simulink model "PalletizeBoxesUsingCobot"  (R2025b)
settings: Solver=FixedStepDiscrete  StartTime=0.0  StopTime=inf  FixedStep=0.01  RelTol=1e-3
PreLoadFcn:
  | EnableGeospatial = false;
  | assignin("base","EnableGeospatial",EnableGeospatial);
  | projectDir = fileparts(which('PalletizeBoxesUsingCobot.slx'));
  | if projectDir == ""
  |     projectDir = pwd;
  | end
  | BoxSet = readtable(fullfile(projectDir,"boxes.xlsx"));
  | assignin("base","BoxSet",BoxSet);
InitFcn:
  | clear boxData boxDataAll boxTable layoutPlan layoutPos layoutYaw layoutH layoutN boxDim boxWeight boxPosition pickPosition boxToEEOffset suctionCenterOffsetCheck maxNumOfBoxes executionActionLog executionActorRegistry
  | projectDir = fileparts(which('PalletizeBoxesUsingCobot.slx'));
  | if projectDir == ""
  |     projectDir = pwd;
  | end
  | disp("Reading Excel from: " + fullfile(projectDir,"boxes.xlsx"));
  | boxTable = readtable(fullfile(projectDir,"boxes.xlsx"));
  | cfg = palletTaskConfig();
  | EnableGeospatial = false;
  | boxDataAll.length = boxTable.L;
  | boxDataAll.width  = boxTable.W;
  | boxDataAll.height = boxTable.H;
  | boxDataAll.weight = boxTable.Mass;
  | if ismember("Type", string(boxTable.Properties.VariableNames)); boxDataAll.type = string(boxTable.Type); end
  | layoutBoxOffset = cfg.layoutBoxOffset;
  | firstExcelID = cfg.firstExcelID;
  | boxData = sliceBoxData(boxDataAll, firstExcelID);
  | nLayoutBoxes = min(cfg.maxLayoutBoxes, numel(boxData.length));
  | boxData.length = boxData.length(1:nLayoutBoxes);
  | boxData.width = boxData.width(1:nLayoutBoxes);
  | boxData.height = boxData.height(1:nLayoutBoxes);
  | boxData.weight = boxData.weight(1:nLayoutBoxes);
  | if isfield(boxData,"type"); boxData.type = boxData.type(1:nLayoutBoxes); end
  | palletDim = cfg.palletDim;
  | palletMargin = cfg.palletMargin;
  | boxGap = cfg.boxGap;
  | palletLoc = cfg.palletLoc;
  | batchSize = cfg.batchSize;
  | layoutPlan = buildLayoutPlanBatch3(boxData, palletDim, palletLoc, batchSize, palletMargin, boxGap);
  | executionPlan = buildBufferExecutionPlan(layoutPlan, cfg);
  | layoutN = numel(layoutPlan);
  | layoutPos = zeros(layoutN,3);
  | layoutYaw = zeros(layoutN,1);
  | layoutH = zeros(layoutN,1);
  | for i = 1:layoutN
  |     layoutPos(i,:) = layoutPlan(i).pos;
  |     layoutYaw(i) = layoutPlan(i).yaw;
  |     layoutH(i) = layoutPlan(i).H;
  | end
  | boxDim = [boxData.length(1); boxData.width(1); boxData.height(1)];
  | boxWeight = boxData.weight(1);
  | boxPosition = cfg.sourceBoxPosition;
  | pickPosition = cfg.pickPosition;
  | boxToEEOffset = [-0.2 0 boxDim(3)/2 + 0.11];
  | suctionCenterOffsetCheck = boxToEEOffset + [0.2 0 0];
  | maxNumOfBoxes = numel(executionPlan);
  | enableSimulinkRRT = false;
  | executionActionLog = zeros(0,4);
  | executionActorRegistry = cell(1,layoutN);
  | rbt = exampleHelperSetUpCobot();
  | assignin("base","boxData",boxData);
  | assignin("base","boxDataAll",boxDataAll);
  | assignin("base","layoutBoxOffset",layoutBoxOffset);
  | assignin("base","firstExcelID",firstExcelID);
  | assignin("base","palletDim",palletDim);
  | assignin("base","palletMargin",palletMargin);
  | assignin("base","boxGap",boxGap);
  | assignin("base","palletLoc",palletLoc);
  | assignin("base","layoutPlan",layoutPlan);
  | assignin("base","executionPlan",executionPlan);
  | assignin("base","layoutMethod","Constructive");
  | assignin("base","batchSize",batchSize);
  | assignin("base","layoutPos",layoutPos);
  | assignin("base","layoutYaw",layoutYaw);
  | assignin("base","layoutH",layoutH);
  | assignin("base","layoutN",layoutN);
  | assignin("base","boxDim",boxDim);
  | assignin("base","boxWeight",boxWeight);
  | assignin("base","boxPosition",boxPosition);
  | assignin("base","pickPosition",pickPosition);
  | assignin("base","boxToEEOffset",boxToEEOffset);
  | assignin("base","suctionCenterOffsetCheck",suctionCenterOffsetCheck);
  | assignin("base","maxNumOfBoxes",maxNumOfBoxes);
  | assignin("base","enableSimulinkRRT",enableSimulinkRRT);
  | assignin("base","executionActionLog",executionActionLog);
  | assignin("base","executionActorRegistry",executionActorRegistry);
  | assignin("base","rbt",rbt);
  | assignin("base","EnableGeospatial",EnableGeospatial);
StartFcn:
  | coder.extrinsic("spawnBox")
  | coder.extrinsic("spawnBufferZone")
  | coder.extrinsic("selectBoxDim")
  | [boxDim, boxWeight] = selectBoxDim(0);
  | boxToEEOffset = [-0.2 0 boxDim(3)/2 + 0.11];
  | suctionCenterOffsetCheck = boxToEEOffset + [0.2 0 0];
  | assignin("base","boxDim",boxDim);
  | assignin("base","boxWeight",boxWeight);
  | assignin("base","boxToEEOffset",boxToEEOffset);
  | assignin("base","suctionCenterOffsetCheck",suctionCenterOffsetCheck);
  | spawnBufferZone()
  | spawnBox(0,boxPosition,boxDim)
StopFcn:
  | try
  |     if exist("executionPlan","var") && ~isempty(executionPlan)
  |         finalizeExecutionAction(numel(executionPlan)-1);
  |     end
  | catch ME
  |     warning("PalletizeBoxes:FinalizeLastAction","%s",ME.message);
  | end
  | disp("Buffer execution simulation stopped.")
libraries: sim3dlib x2, robotcorelib x2, robotmaniplib x2, robotsim3dlib x1, simulink x1
settings Model: PauseTimes=1  Creator=araman  LastModifiedBy=周家易1
settings DebuggingCC: ReadBeforeWriteMsg=DisableAll  WriteAfterWriteMsg=DisableAll  WriteAfterReadMsg=DisableAll  MultiTaskDSMMsg=none
settings ModelReferenceCC: UpdateModelReferenceTargets=IfOutOfDate
settings SFSimCC: SFSimEcho=off

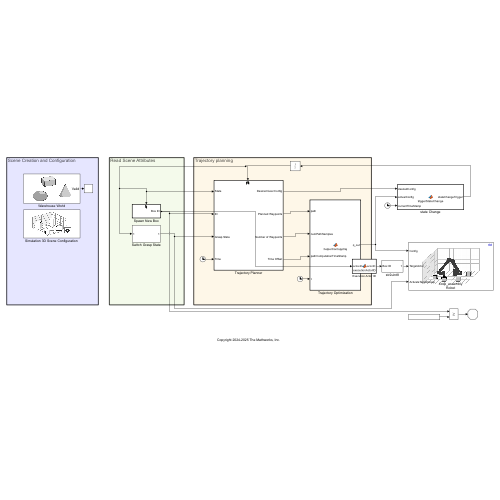
[thumbnail: Simulink's stored preview of the top-level diagram]
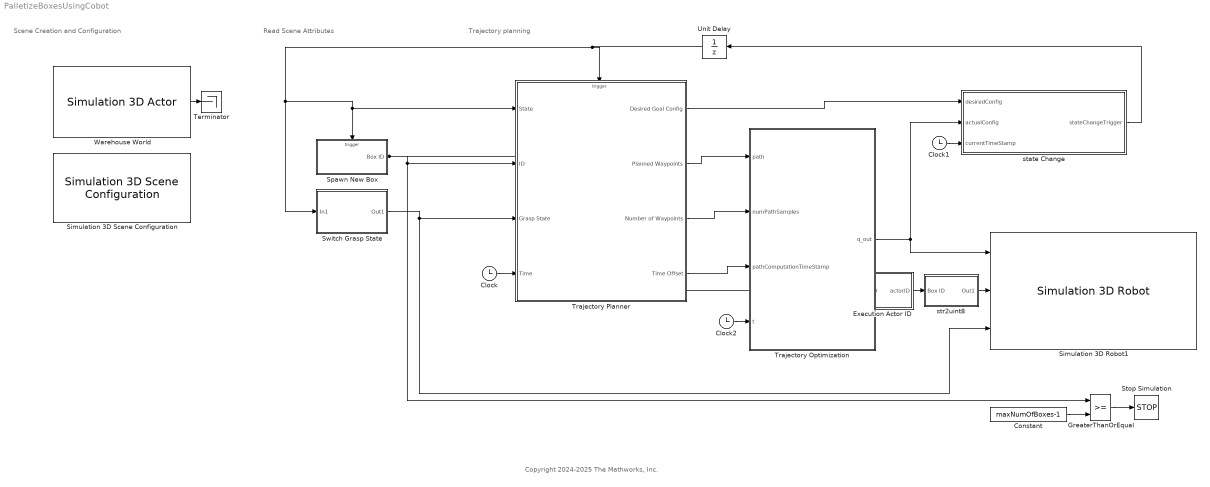
== system PalletizeBoxesUsingCobot ==
  note: Copyright 2024-2025 The Mathworks, Inc.
  note: Trajectory planning
  note: Scene Creation and Configuration
  note: Read Scene Attributes
  Clock : Clock
  Clock1 : Clock
  Clock2 : Clock
  Constant : Constant  Value=maxNumOfBoxes-1
  Execution Actor ID : MATLAB Function  TreatAsAtomicUnit=on
  GreaterThanOrEqual : RelationalOperator  OutDataTypeStr=boolean  RndMeth=Simplest  InputSameDT=off
  Simulation 3D Robot1 : robotsim3dlib/Simulation 3D Robot  actorInputType=RigidBodyTree Object  RigidBodyTree=rbt  ActorName=Robot  existActorChekBox=off  initialTrans=[0 0 0]  initialRot=[0 0 0]  initialConfig="[2.8471   -1.6598    2.1329    4.2393   -1.5708    4.4179]"  EndEffector=4cup_assembly  eeOffsetInpChekBox=off  eeTargetTrans=[0 -0.2 0]  eeTargetRot=[0 0 0]  enableRegionGraspChekBox=off  regionGraspInpChekBox=off  eeTargTransDiff=[0.2 0.2 0.2]  eeTargRotDiff=[0 0 0]  enableVisualVisualization=on  enableCollisionVisualization=off  collisionGeomColor=[0 1 0]  collisionGeomTransp=0.1  inpConfEnbVal=on  inpGraspEnbVal=on  inpTransEnbVal=off  outConfEnbVal=off  outGraspEnbVal=off  outTransEnbVal=off  SampleTime=-1  ActorType=SimulinkVehicle  ID=C  aMode=6  ActorTag=Robot  Mesh=RigidBodyTree
  "Simulation 3D Scene Configuration " : sim3dlib/Simulation 3D Scene Configuration  Priority=0  ProjectFormat=Default Scenes  SceneDesc=Empty scene  ProjectName=D:\matlab2025b\toolbox\shared\sim3d_projects\automotive_project_windows\UE\WindowsNoEditor\VehicleSimulation.exe  ScenePath=/Game/Maps/EmptyScene  EnableOpenDRIVE=off  vehTagList={'Custom';'Robot';'Scene Origin';'Warehouse'}  vehTag=Robot  AttachedCameraRelativeTranslation=[0 0 0]  FreeCameraDefaultInitialTranslation=[-6, 0, 2]  AttachedCameraRelativeRotation=[0 0 0]  FreeCameraDefaultInitialRotation=[0, -15, 0]  ViewpointName=Custom  FreeCameraInitialTranslation=[0, 0, 5]  ViewpointTranslation=[0 0 0]  FreeCameraInitialRotation=[0, -90, 0]  ViewpointRotation=[0 0 0]  OpVisEn=off  Ts=0.02  EnableWindow=on  EnableRemoteAccess=off  EnableWeather=off  SunAzimuth=90  SunAltitude=40.0  EnableGeospatialSun=off  Latitude=0  Longitude=0  Date=2023-01-01  Time=10:30:00  GeoTimeZone=-5.0  SunDaylightSaving=off  wind=1  clouds=10  EnableVolumetricClouds=off  CloudCoverage=0  CloudAltitude=6  fog=0  rain=0  RaindropsEffect=off  SnowDensity=0  EnableGeospatial=off  TilesetSource=Earth terrain  UseTrueOrigin=off  OriginHeight=200  OriginLatitude=40.744652  OriginLongitude=-73.988864  MapStyle=Aerial  AdditionalAssetIDs=[]  UseAdvancedSunSky=off  SolarTime=11  TimeZone=-5  Day=21  Month=9  Year=2022  UseDaylightSavingTime=on  DSTStartDay=10  DSTStartMonth=3  DSTEndDay=3  DSTEndMonth=11  DSTSwitchHour=2  sensorTag=MainCamera2  sensorId=2  sensorName=MainCamera2  mountLoc=Origin  offsetFlag=off  tmountOffset=[0, 0, 0]  rmountOffset=[0, 0, 0]  HorizontalResolution=1280  VerticalResolution=720  HorizontalFOV=60  mountPoint=[0 0 0]  mountOrientation=[0 0 0]  aMode=6  ID=2  GeoTrigger=Inactive  ViewNameList={'Custom'}  ViewTranslationList={'[0 0 5]'}  ViewRotationList={'[0 -90 0]'}
      settings: LibrarySourceBlock=robotsim3dlib/Simulation 3D Scene Configuration
  Spawn New Box : Subsystem  TreatAsAtomicUnit=on
  Stop Simulation : Stop
  Switch Grasp State : Subsystem
  Terminator : Terminator
  Trajectory Optimization : MATLAB Function  TreatAsAtomicUnit=on
  Trajectory Planner : Subsystem
  Unit Delay : UnitDelay  InitialCondition=-1  SampleTime=-1  HasFrameUpgradeWarning=on
  Warehouse World : sim3dlib/Simulation 3D Actor  Priority=1  ActorName=Warehouse  ParentName=Scene Origin  Operation=Create at setup  InitScriptText=|  SampleTime=-1  Translation=single([0 0 0])  Rotation=single([0 0 0])  Scale=single([1 1 1])  aMode=5  ActorTag=Warehouse  ActorType=Sim3dActor  ID=2
      | Plane = sim3d.Actor(ActorName='Plane');
      | Plane.createShape('plane',[5 5 0.1]);
      | Plane.PreciseContacts = true;
      | Plane.Color = [81, 94, 120]/256;
      | add(World,Plane,Actor);
      | 
      | Base = sim3d.Actor('ActorName','collBase');
      | Base.createShape('box',[0.25,0.25,0.5]);
      | Base.Translation = [0,0,0.25];
      | Base.Color = [87, 67, 60]/256;
      | add(World,Base,Actor);
      | 
      | Bench = sim3d.Actor('ActorName','collBench');
      | Bench.createShape('box',[0.8 0.8 0.5]);
      | Bench.Translation = [-0.7 -0.7 0.25];
      | Bench.Color = [87, 67, 60]/256;
      | add(World,Bench,Actor);
      | 
      | Pallet = sim3d.Actor(ActorName='collPallet');
      | add(World,Pallet,Actor)
      | load(Pallet,"PalletEuro.stl",0.001*[1 1 1]);
      | Pallet.Translation = [-1 -0.3 0];
      | Pallet.Collisions = true;
      | Pallet.PreciseContacts = true;
      | PalletDeck = sim3d.Actor(ActorName='PalletDeck');
      | PalletDeck.createShape('box',[0.8 1.2 0.01]);
      | PalletDeck.Translation = [-0.6 0.3 0.139];
      | PalletDeck.Collisions = true;
      | PalletDeck.PreciseContacts = true;
      | PalletDeck.Color = [1 1 1];
      | try, PalletDeck.Opacity = 0; catch, end
      | try, PalletDeck.Transparency = 1; catch, end
      | try, PalletDeck.Visible = false; catch, end
      | add(World,PalletDeck,Actor);
      | 
      | 
      | 
      | 
      | 
      | 
      | 
      | 
      | 
      | 
      | 
      | 
      | 
      | 
      | 
      | 
      | 
      | 
      | 
      | 
      | 
      | 
      | 
      | 
      | 
      | 
      | 
      | Pallet.Collisions = true;
      | Pallet.PreciseContacts = true;
      | Pallet.Collisions = true;
      | Pallet.PreciseContacts = true;
      | Pallet.Collisions = true;
      | Pallet.PreciseContacts = true;
      | Pallet.Collisions = true;
      | Pallet.PreciseContacts = true;
      | Pallet.Collisions = true;
      | Pallet.PreciseContacts = true;
      | Pallet.Collisions = true;
      | Pallet.PreciseContacts = true;
      | Pallet.Collisions = true;
      | Pallet.PreciseContacts = true;
      | Pallet.Collisions = true;
      | Pallet.PreciseContacts = true;
      | Pallet.Collisions = true;
      | Pallet.PreciseContacts = true;
      | Pallet.Collisions = true;
      | Pallet.PreciseContacts = true;
      | Pallet.Collisions = true;
      | Pallet.PreciseContacts = true;
      | Pallet.Collisions = true;
      | Pallet.PreciseContacts = true;
      | Pallet.Collisions = true;
      | Pallet.PreciseContacts = true;
  state Change : MATLAB Function  TreatAsAtomicUnit=on
  str2uint8 : Subsystem
  wires:
  Warehouse World/1 -> Terminator/1
  Unit Delay/1 -> Switch Grasp State/1(In1), Spawn New Box/Trigger, Trajectory Planner/1(State), Trajectory Planner/Trigger
  Clock/1 -> Trajectory Planner/4(Time)
  Trajectory Planner/2(Planned Waypoints) -> Trajectory Optimization/1(path)
  Trajectory Planner/3(Number of Waypoints) -> Trajectory Optimization/2(numPathSamples)
  Trajectory Planner/4(Time Offset) -> Trajectory Optimization/3(pathComputationTimeStamp)
  Trajectory Planner/1(Desired Goal Config) -> state Change/1(desiredConfig)
  Spawn New Box/1(Box ID) -> Trajectory Planner/2(ID), GreaterThanOrEqual/1, Execution Actor ID/1(actionID)
  Clock1/1 -> state Change/3(currentTimeStamp)
  state Change/1(stateChangeTrigger) -> Unit Delay/1
  Clock2/1 -> Trajectory Optimization/4(t)
  Switch Grasp State/1(Out1) -> Simulation 3D Robot1/3, Trajectory Planner/3(Grasp State)
  Trajectory Optimization/1(q_out) -> Simulation 3D Robot1/1, state Change/2(actualConfig)
  Constant/1 -> GreaterThanOrEqual/2
  GreaterThanOrEqual/1 -> Stop Simulation/1
  str2uint8/1(Out1) -> Simulation 3D Robot1/2
  Execution Actor ID/1(actorID) -> str2uint8/1(Box ID)

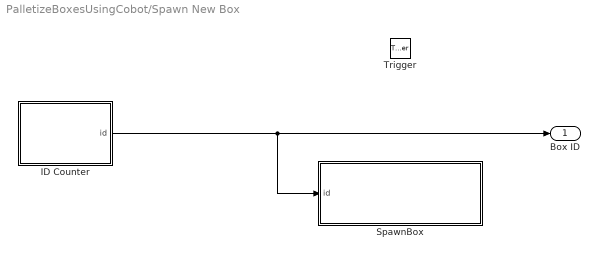
== system PalletizeBoxesUsingCobot/Spawn New Box ==
  Trigger : TriggerPort  TriggerType=falling  VariantControl=(inherit)
  ID Counter : Subsystem
  "SpawnBox " : MATLAB Function  TreatAsAtomicUnit=on
  Box ID : Outport
  wires:
  ID Counter/1(id) -> "SpawnBox "/1(id), Box ID/1

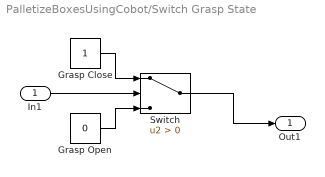
== system PalletizeBoxesUsingCobot/Switch Grasp State ==
  In1 : Inport
  Grasp Close : Constant  OutDataTypeStr=boolean
  Grasp Open : Constant  Value=0  OutDataTypeStr=boolean
  Switch : Switch  Criteria=u2 > Threshold  SaturateOnIntegerOverflow=off  InputSameDT=off
  Out1 : Outport
  wires:
  Grasp Close/1 -> Switch/1
  Switch/1 -> Out1/1
  Grasp Open/1 -> Switch/3
  In1/1 -> Switch/2

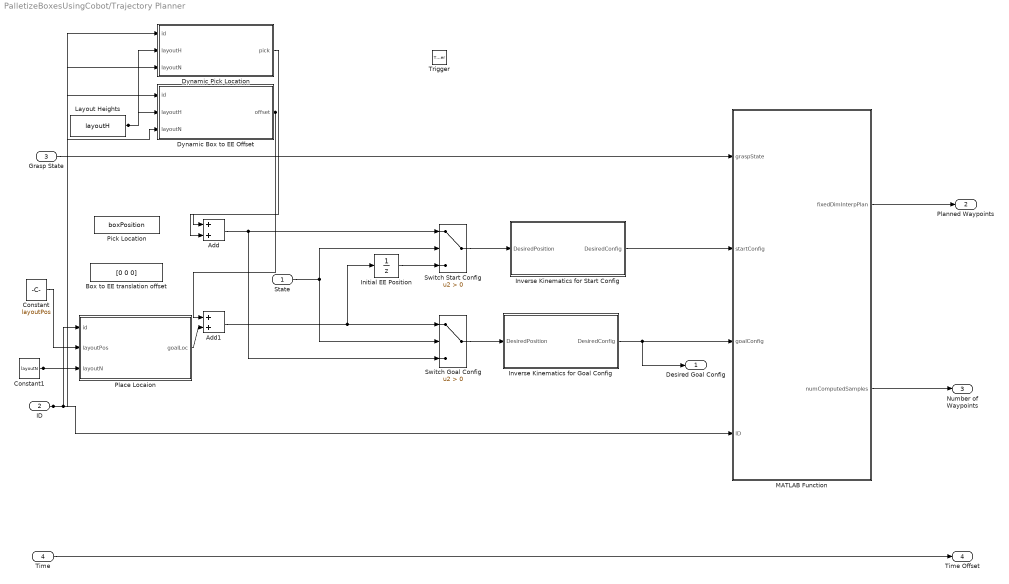
== system PalletizeBoxesUsingCobot/Trajectory Planner ==
  State : Inport
  ID : Inport  Port=2
  Grasp State : Inport  Port=3
  Time : Inport  Port=4
  Trigger : TriggerPort  TriggerType=either  VariantControl=(inherit)  OutputDataType=double  InitialTriggerSignalState=zero  PortDimensions=1
  Add : Sum
  Add1 : Sum
  Box to EE translation offset : Constant  Value=[0 0 0]  VectorParams1D=off
  Constant : Constant  Value=layoutPos
  Constant1 : Constant  Value=layoutN
  Dynamic Box to EE Offset : MATLAB Function  TreatAsAtomicUnit=on
  Dynamic Pick Location : MATLAB Function  TreatAsAtomicUnit=on
  Initial EE Position : UnitDelay  InitialCondition=[-0.6 0 0.8]  SampleTime=-1  HasFrameUpgradeWarning=on
  Inverse Kinematics for Goal Config : Subsystem
  Inverse Kinematics for Start Config : Subsystem
  Layout Heights : Constant  Value=layoutH
  MATLAB Function : MATLAB Function  TreatAsAtomicUnit=on
  Pick Location : Constant  Value=boxPosition  VectorParams1D=off
  Place Locaion : MATLAB Function  TreatAsAtomicUnit=on
  Switch Goal Config : Switch  Criteria=u2 > Threshold  SaturateOnIntegerOverflow=off  InputSameDT=off
  Switch Start Config : Switch  Criteria=u2 > Threshold  SaturateOnIntegerOverflow=off  InputSameDT=off
  Desired Goal Config : Outport
  Planned Waypoints : Outport  Port=2
  Number of Waypoints : Outport  Port=3
  Time Offset : Outport  Port=4
  wires:
  MATLAB Function/1(fixedDimInterpPlan) -> Planned Waypoints/1
  MATLAB Function/2(numComputedSamples) -> Number of Waypoints/1
  Inverse Kinematics for Start Config/1(DesiredConfig) -> MATLAB Function/2(startConfig)
  Inverse Kinematics for Goal Config/1(DesiredConfig) -> MATLAB Function/3(goalConfig), Desired Goal Config/1
  Time/1 -> Time Offset/1
  Switch Start Config/1 -> Inverse Kinematics for Start Config/1(DesiredPosition)
  Initial EE Position/1 -> Switch Start Config/3
  Switch Goal Config/1 -> Inverse Kinematics for Goal Config/1(DesiredPosition)
  Add/1 -> Switch Start Config/1, Switch Goal Config/3
  State/1 -> Switch Start Config/2, Switch Goal Config/2
  Grasp State/1 -> MATLAB Function/1(graspState)
  ID/1 -> MATLAB Function/4(ID), Place Locaion/1(id), Dynamic Box to EE Offset/1(id), Dynamic Pick Location/1(id)
  Place Locaion/1(goalLoc) -> Add1/2
  Add1/1 -> Initial EE Position/1, Switch Goal Config/1
  Constant/1 -> Place Locaion/2(layoutPos)
  Constant1/1 -> Place Locaion/3(layoutN), Dynamic Box to EE Offset/3(layoutN), Dynamic Pick Location/3(layoutN)
  Layout Heights/1 -> Dynamic Box to EE Offset/2(layoutH), Dynamic Pick Location/2(layoutH)
  Dynamic Box to EE Offset/1(offset) -> Add/2, Add1/1
  Dynamic Pick Location/1(pick) -> Add/1

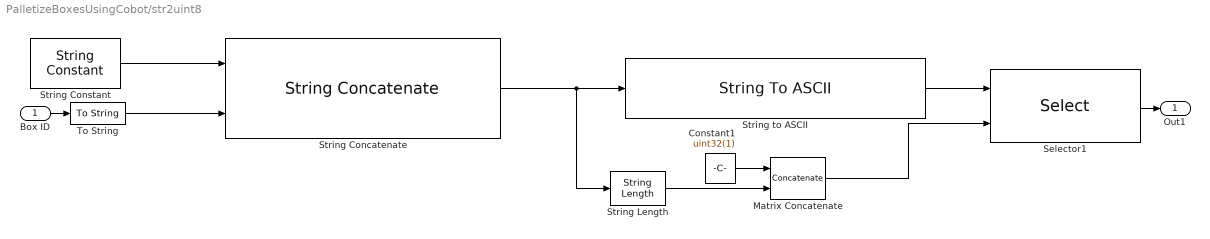
== system PalletizeBoxesUsingCobot/str2uint8 ==
  Box ID : Inport
  Constant1 : Constant  Value=uint32(1)
  Matrix Concatenate : Concatenate  ConcatenateDimension=2
  Selector1 : Selector  InputPortWidth=12  IndexOptions=Starting and ending indices (port)  Indices=[1 3]  OutputSizes=1
  String Concatenate : StringConcatenate
  String Constant : StringConstant  String="\"collBox\""
  String Length : StringLength
  String to ASCII : StringToASCII  OutputVectorSize=12
  To String : ToString
  Out1 : Outport
  wires:
  String Constant/1 -> String Concatenate/1
  Constant1/1 -> Matrix Concatenate/1
  String Length/1 -> Matrix Concatenate/2
  String Concatenate/1 -> String Length/1, String to ASCII/1
  Box ID/1 -> To String/1
  Matrix Concatenate/1 -> Selector1/2
  String to ASCII/1 -> Selector1/1
  To String/1 -> String Concatenate/2
  Selector1/1 -> Out1/1

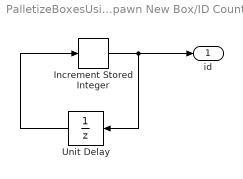
== system PalletizeBoxesUsingCobot/Spawn New Box/ID Counter ==
  Increment Stored Integer : simulink/Additional Math & Discrete/Additional Math: Increment - Decrement/Increment Stored Integer
  Unit Delay : UnitDelay  SampleTime=-1  HasFrameUpgradeWarning=on
  id : Outport
  wires:
  Increment Stored Integer/1 -> id/1, Unit Delay/1
  Unit Delay/1 -> Increment Stored Integer/1

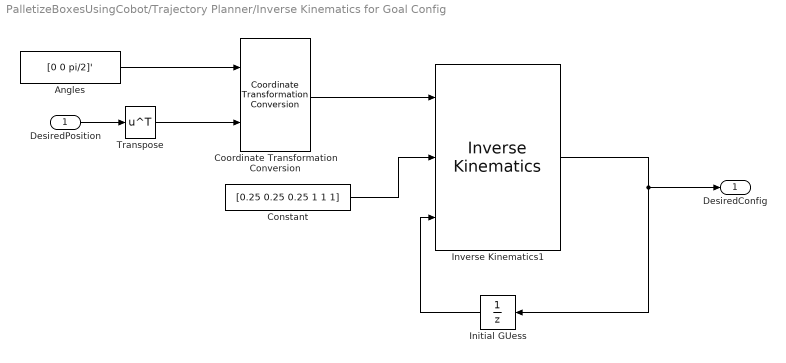
== system PalletizeBoxesUsingCobot/Trajectory Planner/Inverse Kinematics for Goal Config ==
  DesiredPosition : Inport
  Angles : Constant  Value=[0 0 pi/2]'  VectorParams1D=off
  Constant : Constant  Value=[0.25 0.25 0.25 1 1 1]
  Coordinate Transformation Conversion : robotcorelib/Coordinate Transformation Conversion  InputRepresentation=Euler Angles  InputEulerSequence=ZYX  ShowTrVecInputPort=on  OutputRepresentation=Homogeneous Transformation  OutputEulerSequence=ZYX  ShowTrVecOutputPort=on  SimulateUsing=Interpreted execution
  Initial GUess : UnitDelay  InitialCondition="[2.8471   -1.6598    2.1329    4.2393   -1.5708    4.4179]'"  SampleTime=-1  HasFrameUpgradeWarning=on
  Inverse Kinematics1 : robotmaniplib/Inverse Kinematics  RigidBodyTree=rbt  EndEffector=4cup_assembly  ShowInfo=off  SolverName=BFGS Gradient Projection  EnforceJointLimits=on  MaxIterations=40  MaxTime=10  GradientTolerance=1e-7  SolutionTolerance=1e-6  StepTolerance=1e-14  ConstraintTolerance=1e-6  ErrorChangeTolerance=1e-12  UseErrorDamping=on  DampingBias=0.0025  SimulateUsing=Code generation
  Transpose : Math  Operator=transpose
  DesiredConfig : Outport
  wires:
  Constant/1 -> Inverse Kinematics1/2
  Coordinate Transformation Conversion/1 -> Inverse Kinematics1/1
  DesiredPosition/1 -> Transpose/1
  Initial GUess/1 -> Inverse Kinematics1/3
  Inverse Kinematics1/1 -> Initial GUess/1, DesiredConfig/1
  Transpose/1 -> Coordinate Transformation Conversion/2
  Angles/1 -> Coordinate Transformation Conversion/1

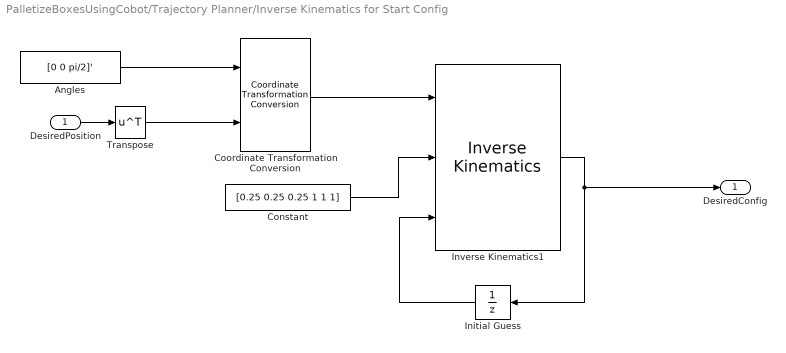
== system PalletizeBoxesUsingCobot/Trajectory Planner/Inverse Kinematics for Start Config ==
  DesiredPosition : Inport
  Angles : Constant  Value=[0 0 pi/2]'  VectorParams1D=off
  Constant : Constant  Value=[0.25 0.25 0.25 1 1 1]
  Coordinate Transformation Conversion : robotcorelib/Coordinate Transformation Conversion  InputRepresentation=Euler Angles  InputEulerSequence=ZYX  ShowTrVecInputPort=on  OutputRepresentation=Homogeneous Transformation  OutputEulerSequence=ZYX  ShowTrVecOutputPort=on  SimulateUsing=Interpreted execution
  Initial Guess : UnitDelay  InitialCondition="[-0.0724   -0.8022    1.6836    3.8   -1.5708    1.3514]'"  SampleTime=-1  HasFrameUpgradeWarning=on
  Inverse Kinematics1 : robotmaniplib/Inverse Kinematics  RigidBodyTree=rbt  EndEffector=4cup_assembly  ShowInfo=off  SolverName=BFGS Gradient Projection  EnforceJointLimits=on  MaxIterations=40  MaxTime=10  GradientTolerance=1e-7  SolutionTolerance=1e-6  StepTolerance=1e-14  ConstraintTolerance=1e-6  ErrorChangeTolerance=1e-12  UseErrorDamping=on  DampingBias=0.0025  SimulateUsing=Code generation
  Transpose : Math  Operator=transpose
  DesiredConfig : Outport
  wires:
  Constant/1 -> Inverse Kinematics1/2
  Angles/1 -> Coordinate Transformation Conversion/1
  Inverse Kinematics1/1 -> DesiredConfig/1, Initial Guess/1
  Initial Guess/1 -> Inverse Kinematics1/3
  Coordinate Transformation Conversion/1 -> Inverse Kinematics1/1
  DesiredPosition/1 -> Transpose/1
  Transpose/1 -> Coordinate Transformation Conversion/2

== matlab function PalletizeBoxesUsingCobot/Trajectory Planner/MATLAB Function ==
  data: graspState input; startConfig input; fixedDimInterpPlan output size=[6,200]; goalConfig input; ID input; numComputedSamples output; boxPosition parameter; boxDim parameter; maxNumOfBoxes parameter
function [fixedDimInterpPlan,numComputedSamples] = helperPathPanning(graspState, startConfig,goalConfig,ID,boxPosition, boxDim, maxNumOfBoxes)
%#codegen
fixedDimInterpPlan = zeros(6, 200);
numComputedSamples = 0;
coder.extrinsic("exampleHelperManipulatorRRT");
[fixedDimInterpPlan,numComputedSamples] = exampleHelperManipulatorRRT(graspState, startConfig,goalConfig,ID,boxPosition, boxDim, maxNumOfBoxes);
end

== matlab function PalletizeBoxesUsingCobot/state Change ==
  data: desiredConfig input; stateChangeTrigger output; actualConfig input; currentTimeStamp input
function stateChangeTrigger = triggerStateChange(desiredConfig,actualConfig,currentTimeStamp)
%#codegen
tol=0.06; simTimeStep=0.02; maxStateDuration=8.0;
persistent stateChange timeAtStateChange actionCount
if isempty(stateChange)
    stateChange=-1; timeAtStateChange=0; actionCount=0;
end
err=sqrt(sum((desiredConfig-actualConfig).^2));
heldLongEnough=(currentTimeStamp-timeAtStateChange)>simTimeStep;
timedOut=(currentTimeStamp-timeAtStateChange)>maxStateDuration;
if (err<tol || timedOut) && heldLongEnough
    switch stateChange
        case -1
            stateChange=1;
        case 1
            stateChange=-1;
            actionCount=actionCount+1;
    end
    timeAtStateChange=currentTimeStamp;
end
stateChangeTrigger=stateChange;
end

== matlab function PalletizeBoxesUsingCobot/Spawn New Box/SpawnBox  ==
  data: id input; boxPosition parameter; boxDim parameter
function spawnBoxOnBench(id, boxPosition, boxDim)
%#codegen
coder.extrinsic('selectBoxDim');
[boxDim, ~] = selectBoxDim(double(id));
coder.extrinsic('spawnExecutionActionBox');
spawnExecutionActionBox(id, boxPosition, boxDim);
end

== matlab function PalletizeBoxesUsingCobot/Trajectory Optimization ==
  data: path input size=[6,200]; numPathSamples input; pathComputationTimeStamp input; t input; q_out output
function q_out = helperContopptraj(path, numPathSamples, pathComputationTimeStamp, t)

VELLIM = repmat([-10  10], 6, 1);   % Velocity limits for trajectory
ACCELLIM = repmat([-15 15], 6, 1); % Acceleration limits for trajectory

% Store the last time at which the path was computed as a persistent
% variable. This allows the function to detect changes
persistent prevPathComputationTime qSolve tSolve
if isempty(prevPathComputationTime)
    prevPathComputationTime = -1;
end
if isempty(qSolve)
    qSolve = repmat([2.8471   -1.6598    2.1329    4.2393   -1.5708    4.4179]',1,500);
    tSolve = linspace(0,2,500);
end

% Compute a time constrained trajectory with contoptraj
if (pathComputationTimeStamp ~= prevPathComputationTime) && (numPathSamples > 0)
    [qSolve,~,~,tSolve] = contopptraj(path(:,1:numPathSamples),VELLIM,ACCELLIM,NumSamples=100);
end
%if (pathComputationTimeStamp ~= prevPathComputationTime) && (numPathSamples > 0)
%    qSolve(:,1:numPathSamples) = path(:,1:numPathSamples);
%end

% Compute the output at an instant in time t. Because contopptraj defines
% the time stamp relative to a clock that begins at zero, subtract the time
% stamp at computation time from the current time.
q_out = zeros(6,1);

maxTime = max(tSolve);
queryTime = t - pathComputationTimeStamp;
if queryTime == 0
    q_out(:) = qSolve(:,1);
elseif queryTime <= maxTime
    % Use linear interpolation to approximate the reference trajectory
    % inside the time range for which it is defined
    q_out(:) = interp1(tSolve,qSolve',queryTime);
else
    % After the trajectory end is reached, if no new trajectory is
    % computed, hold the last value
    q_out(:) = qSolve(:,end);
end

% Update the stored path computation time stamp
prevPathComputationTime = pathComputationTimeStamp;

end

== matlab function PalletizeBoxesUsingCobot/Trajectory Planner/Dynamic Box to EE Offset ==
  data: id input; offset output; layoutH input; layoutN input
function offset = dynamicBoxToEEOffset(id, layoutH, layoutN)
%#codegen
offset = zeros(1,3);
boxDim = zeros(3,1);
coder.extrinsic('selectBoxDim');
[boxDim,~] = selectBoxDim(double(id));
offset(1) = -0.2;
offset(3) = double(boxDim(3))/2 + 0.11;
end

== matlab function PalletizeBoxesUsingCobot/Trajectory Planner/Dynamic Pick Location ==
  data: id input; pick output; layoutH input; layoutN input
function pick = dynamicPickLocation(id, layoutH, layoutN)
%#codegen
pick = zeros(1,3);
coder.extrinsic('getExecutionPickLocation');
pick = getExecutionPickLocation(double(id));
end

== matlab function PalletizeBoxesUsingCobot/Execution Actor ID ==
  data: actionID input; actorID output
function actorID = executionActorID(actionID)
%#codegen
actorID = 0;
coder.extrinsic('getExecutionActorID');
actorID = getExecutionActorID(double(actionID));
end

== matlab function PalletizeBoxesUsingCobot/Trajectory Planner/Place Locaion ==
  data: id input; goalLoc output; layoutPos input; layoutN input
function goalLoc = getGoalOnPallet(id, layoutPos, layoutN)
%#codegen
goalLoc = zeros(1,3);
coder.extrinsic('getExecutionPlaceLocation');
goalLoc = getExecutionPlaceLocation(double(id));
end
